simulink subsystem "gearsBlock"  (R2024a)
settings: Solver=VariableStepAuto  StartTime=0.0  StopTime=10.0  RelTol=1e-3
libraries: fl_lib x4
settings Model: Creator=malemi  LastModifiedBy=mattrich

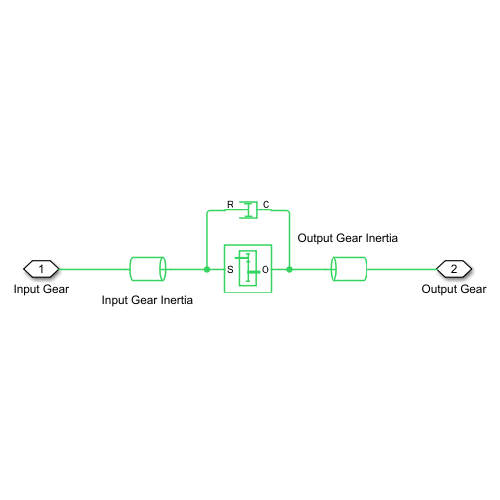
[thumbnail: Simulink's stored preview of the top-level diagram]
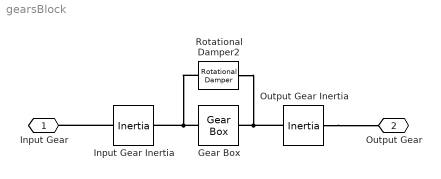
== system gearsBlock ==
  Gear Box : fl_lib/Mechanical/Mechanisms/Gear Box  ratio=2  t_in_specify=off  t_in_priority=None  t_in=0 N*m  t_in_nominal_specify=off  t_in_nominal_value=1  t_in_nominal_unit=N*m  t_out_specify=off  t_out_priority=None  t_out=0 N*m  t_out_nominal_specify=off  t_out_nominal_value=1  t_out_nominal_unit=N*m
  Input Gear Inertia : fl_lib/Mechanical/Rotational Elements/Inertia  inertia=6 cm^2*g  num_ports=foundation.enum.numPorts2.two  w_specify=off  w_priority=High  w=0 rad/s  w_nominal_specify=off  w_nominal_value=1  w_nominal_unit=rad/s  t_specify=off  t_priority=None  t=0 N*m  t_nominal_specify=off  t_nominal_value=1  t_nominal_unit=N*m
      settings: InternalSimscapePortConfiguration="{\"Bottom\":[],\"Left\":[{\"id\":\"I\",\"label\":\"\",\"type\":\"foundation.mechanical.rotational.rotational\"}],\"Right\":[{\"id\":\"J\",\"label\":\"\",\"type\":\"foundation.mechanical.rotational.rotational\"}],\"Top\":[]}"
  Output Gear Inertia : fl_lib/Mechanical/Rotational Elements/Inertia  inertia=100 cm^2*g  num_ports=foundation.enum.numPorts2.two  w_specify=off  w_priority=High  w=0 rad/s  w_nominal_specify=off  w_nominal_value=1  w_nominal_unit=rad/s  t_specify=off  t_priority=None  t=0 N*m  t_nominal_specify=off  t_nominal_value=1  t_nominal_unit=N*m
      settings: InternalSimscapePortConfiguration="{\"Bottom\":[],\"Left\":[{\"id\":\"I\",\"label\":\"\",\"type\":\"foundation.mechanical.rotational.rotational\"}],\"Right\":[{\"id\":\"J\",\"label\":\"\",\"type\":\"foundation.mechanical.rotational.rotational\"}],\"Top\":[]}"
  Rotational Damper2 : fl_lib/Mechanical/Rotational Elements/Rotational Damper  D=0.0001 N*m*s/rad  w_specify=off  w_priority=None  w=0 rad/s  w_nominal_specify=off  w_nominal_value=1  w_nominal_unit=rad/s  t_specify=off  t_priority=None  t=0 N*m  t_nominal_specify=off  t_nominal_value=1  t_nominal_unit=N*m
  Input Gear : PMIOPort  Side=Left
  Output Gear : PMIOPort  Port=2  Side=Right
  connections:
  Rotational Damper2/LConn1 -- Input Gear Inertia/LConn1 -- Gear Box/LConn1
  Output Gear Inertia/LConn1 -- Gear Box/RConn1 -- Rotational Damper2/RConn1
  Input Gear Inertia/RConn1 -- Input Gear/RConn1
  Output Gear Inertia/RConn1 -- Output Gear/RConn1
